simulink model "torque_est_code_source"  (R2024b)
settings: Solver=VariableStepAuto  StartTime=0.0  StopTime=20  RelTol=1e-3
model workspace (MAT data in the model file):
  Efficiency = 106.795164671
  Ktau = 0.0593933626833
  Kw = 0.000707222843993
  To = 0.029588829084
  alfa = 1.29
undefined symbols (not defined in the file or in its folder): DiscIntNeverNeededParam
settings Model: Creator=ascalzo  LastModifiedBy=upattacini
settings OptimizationCC: DefaultParameterBehavior=Inlined  UseDivisionForNetSlopeComputation=on  GainParamInheritBuiltInType=on  UseFloatMulNetSlope=on  InlineInvariantSignals=on  PassReuseOutputArgsAs=Individual arguments  ZeroExternalMemoryAtStartup=off  ZeroInternalMemoryAtStartup=off  NoFixptDivByZeroProtection=on  EfficientFloat2IntCast=on  LifeSpan=1  OptimizeBlockOrder=speed  DifferentSizesBufferReuse=on  EfficientTunableParamExpr=on
settings DebuggingCC: ParameterTunabilityLossMsg=error
settings HardwareCC: ProdBitPerPointer=32  ProdBitPerSizeT=32  ProdBitPerPtrDiffT=32  ProdLargestAtomicInteger=Long  ProdLargestAtomicFloat=Double  ProdWordSize=32  ProdLongLongMode=on  ProdHWDeviceType=ARM Compatible->ARM Cortex-M
settings SFSimCC: MATLABDynamicMemAlloc=off
settings RTWCC: Description=Embedded Coder  SystemTargetFile=ert.tlc  GenCodeOnly=on  TemplateMakefile=ert_default_tmf  TargetLang=C++  GPUComputeCapability=3.5
settings CodeAppCC: ForceParamTrailComments=on  IgnoreCustomStorageClasses=off  OperatorAnnotations=on  SimulinkDataObjDesc=on  SFDataObjDesc=on  CustomSymbolStrGlobalVar=rt$N$M  CustomSymbolStrType=$N$M  CustomSymbolStrFcn=$N$M$F  CustomSymbolStrMacro=$N$M  InsertBlockDesc=on
settings ERTTargetCC: TargetLangStandard=C++11 (ISO)  CodeReplacementLibrary=ARM Cortex-M  GenerateSampleERTMain=on  IncludeMdlTerminateFcn=off  CombineSignalStateStructs=on  CodeInterfacePackaging=C++ class  SupportComplex=off  SupportNonInlinedSFcns=on  RootIOFormat=Structure reference  ERTCustomFileTemplate=example_file_process.tlc  ERTFilePackagingFormat=CompactWithDataFile  DynamicArrayContainerType=coder::array

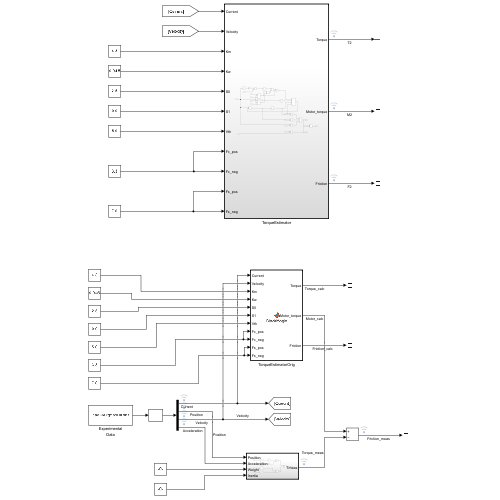
[thumbnail: Simulink's stored preview of the top-level diagram]
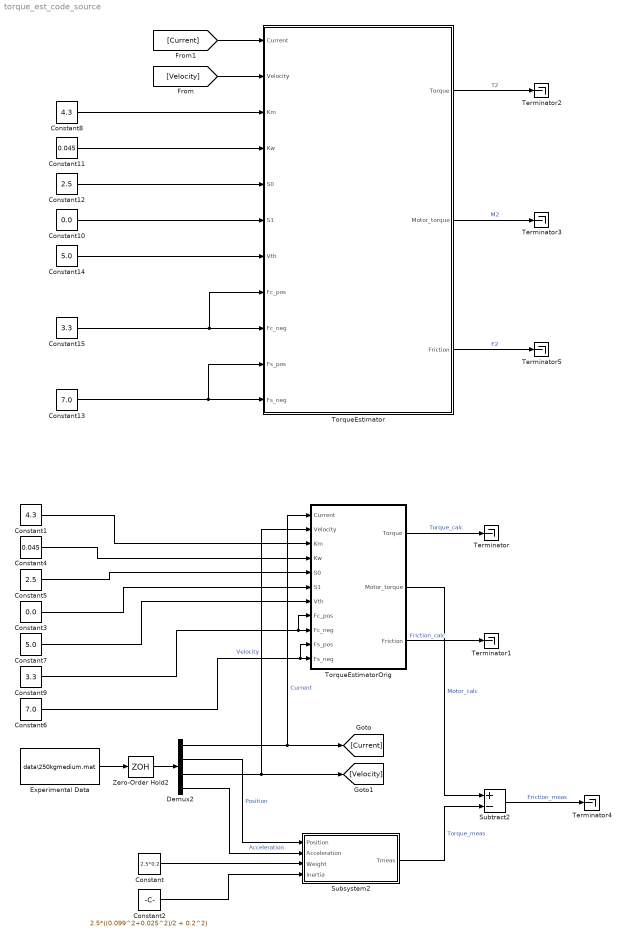
== system torque_est_code_source ==
  Constant : Constant  Value=2.5*0.2
  Constant1 : Constant  Value=4.3
  Constant10 : Constant  Value=0.0
  Constant11 : Constant  Value=0.045
  Constant12 : Constant  Value=2.5
  Constant13 : Constant  Value=7.0
  Constant14 : Constant  Value=5.0
  Constant15 : Constant  Value=3.3
  Constant2 : Constant  Value=2.5*((0.099^2+0.025^2)/2 + 0.2^2)
  Constant3 : Constant  Value=0.0
  Constant4 : Constant  Value=0.045
  Constant5 : Constant  Value=2.5
  Constant6 : Constant  Value=7.0
  Constant7 : Constant  Value=5.0
  Constant8 : Constant  Value=4.3
  Constant9 : Constant  Value=3.3
  Demux2 : Demux
  Experimental Data : FromFile  FileName=data\250kgmedium.mat  SampleTime=0.001  InterpolationWithinTimeRange=Zero order hold
  Subsystem2 : Subsystem  TreatAsAtomicUnit=on
  Subtract2 : Sum  Inputs=+-
  Terminator{,1..5} (6 alike) : Terminator
  TorqueEstimator : Subsystem  TreatAsAtomicUnit=on
  TorqueEstimatorOrig : MATLAB Function  TreatAsAtomicUnit=on
  Zero-Order Hold2 : ZeroOrderHold  SampleTime=0.001
  wires:
  Subtract2/1 -> Terminator4/1  "Friction_meas"
  Experimental Data/1 -> Zero-Order Hold2/1
  Demux2/3 -> [Velocity], TorqueEstimatorOrig/2(Velocity)  "Velocity"
  Zero-Order Hold2/1 -> Demux2/1
  Demux2/4 -> Subsystem2/2(Acceleration)  "Acceleration"
  Demux2/2 -> Subsystem2/1(Position)  "Position"
  Constant/1 -> Subsystem2/3(Weight)
  Constant2/1 -> Subsystem2/4(Inertia)
  Demux2/1 -> [Current], TorqueEstimatorOrig/1(Current)  "Current"
  Subsystem2/1(Tmeas) -> Subtract2/2  "Torque_meas"
  TorqueEstimatorOrig/2(Motor_torque) -> Subtract2/1  "Motor_calc"
  TorqueEstimatorOrig/1(Torque) -> Terminator/1  "Torque_calc"
  TorqueEstimatorOrig/3(Friction) -> Terminator1/1  "Friction_calc"
  Constant1/1 -> TorqueEstimatorOrig/3(Km)
  Constant3/1 -> TorqueEstimatorOrig/6(S1)
  Constant4/1 -> TorqueEstimatorOrig/4(Kw)
  Constant5/1 -> TorqueEstimatorOrig/5(S0)
  Constant6/1 -> TorqueEstimatorOrig/11(Fs_neg), TorqueEstimatorOrig/10(Fs_pos)
  Constant7/1 -> TorqueEstimatorOrig/7(Vth)
  Constant9/1 -> TorqueEstimatorOrig/8(Fc_pos), TorqueEstimatorOrig/9(Fc_neg)
  [Velocity] -> TorqueEstimator/2(Velocity)
  [Current] -> TorqueEstimator/1(Current)
  Constant10/1 -> TorqueEstimator/6(S1)
  Constant15/1 -> TorqueEstimator/8(Fc_pos), TorqueEstimator/9(Fc_neg)
  Constant12/1 -> TorqueEstimator/5(S0)
  Constant14/1 -> TorqueEstimator/7(Vth)
  Constant11/1 -> TorqueEstimator/4(Kw)
  Constant13/1 -> TorqueEstimator/11(Fs_neg), TorqueEstimator/10(Fs_pos)
  Constant8/1 -> TorqueEstimator/3(Km)
  TorqueEstimator/1(Torque) -> Terminator2/1  "T2"
  TorqueEstimator/2(Motor_torque) -> Terminator3/1  "M2"
  TorqueEstimator/3(Friction) -> Terminator5/1  "F2"

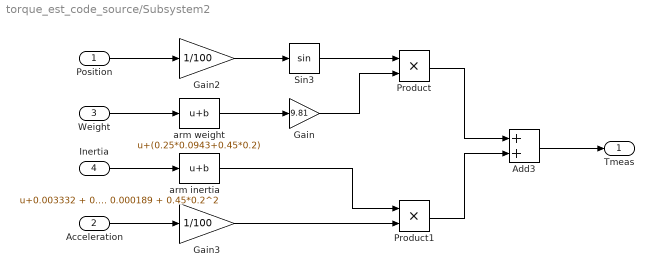
== system torque_est_code_source/Subsystem2 ==
  Position : Inport
  Acceleration : Inport  Port=2
  Weight : Inport  Port=3
  Inertia : Inport  Port=4
  Add3 : Sum
  Gain : Gain  Gain=9.81
  Gain2 : Gain  Gain=1/100
  Gain3 : Gain  Gain=1/100
  Product : Product
  Product1 : Product
  Sin3 : Trigonometry
  arm inertia : Bias  Bias=0.003332 + 0.000021 + 0.000001185 + 0.000189 + 0.45*0.2^2  SaturateOnIntegerOverflow=off
  arm weight : Bias  Bias=(0.25*0.0943+0.45*0.2)  SaturateOnIntegerOverflow=off
  Tmeas : Outport
  wires:
  Product/1 -> Add3/1
  Gain2/1 -> Sin3/1
  Sin3/1 -> Product/1
  Add3/1 -> Tmeas/1
  Gain3/1 -> Product1/2
  Acceleration/1 -> Gain3/1
  Position/1 -> Gain2/1
  Weight/1 -> arm weight/1
  Product1/1 -> Add3/2
  Inertia/1 -> arm inertia/1
  arm weight/1 -> Gain/1
  arm inertia/1 -> Product1/1
  Gain/1 -> Product/2

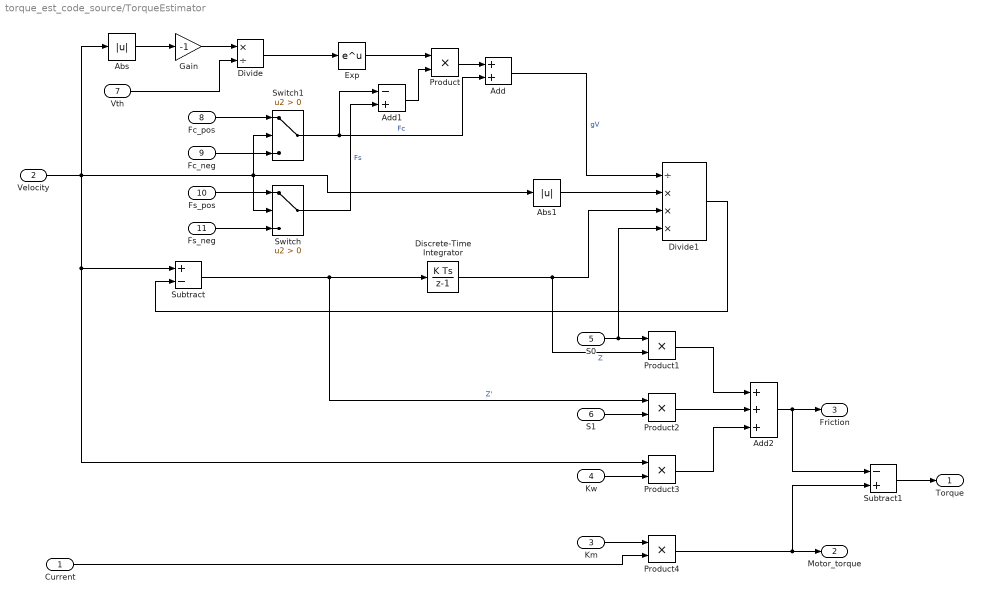
== system torque_est_code_source/TorqueEstimator ==
  Current : Inport
  Velocity : Inport  Port=2
  Km : Inport  Port=3
  Kw : Inport  Port=4
  S0 : Inport  Port=5
  S1 : Inport  Port=6
  Vth : Inport  Port=7
  Fc_pos : Inport  Port=8
  Fc_neg : Inport  Port=9
  Fs_pos : Inport  Port=10
  Fs_neg : Inport  Port=11
  Abs : Abs  SaturateOnIntegerOverflow=off
  Abs1 : Abs  SaturateOnIntegerOverflow=off
  Add : Sum
  Add1 : Sum  Inputs=-+
  Add2 : Sum  Inputs=+++
  Discrete-Time Integrator : DiscreteIntegrator  SampleTime=-1  ICPrevOutput=DiscIntNeverNeededParam  ICPrevScaledInput=DiscIntNeverNeededParam
  Divide : Product  Inputs=*/
  Divide1 : Product  Inputs=/***
  Exp : Math
  Gain : Gain  Gain=-1
  Product{,1..4} (5 alike) : Product
  Subtract : Sum  Inputs=+-
  Subtract1 : Sum  Inputs=-+
  Switch : Switch  Criteria=u2 > Threshold  SaturateOnIntegerOverflow=off  InputSameDT=off
  Switch1 : Switch  Criteria=u2 > Threshold  SaturateOnIntegerOverflow=off  InputSameDT=off
  Torque : Outport
  Motor_torque : Outport  Port=2
  Friction : Outport  Port=3
  wires:
  Fs_pos/1 -> Switch/1
  Kw/1 -> Product3/2
  Abs1/1 -> Divide1/2
  S0/1 -> Divide1/4, Product1/1
  Product2/1 -> Add2/2
  Velocity/1 -> Abs1/1, Switch/2, Switch1/2, Product3/1, Subtract/1, Abs/1
  Fs_neg/1 -> Switch/3
  Switch1/1 -> Add/2, Add1/1  "Fc"
  Subtract/1 -> Discrete-Time Integrator/1, Product2/1  "Z'"
  Exp/1 -> Product/1
  Discrete-Time Integrator/1 -> Divide1/3, Product1/2  "Z"
  Fc_neg/1 -> Switch1/3
  Fc_pos/1 -> Switch1/1
  Gain/1 -> Divide/1
  Product1/1 -> Add2/1
  Abs/1 -> Gain/1
  Product3/1 -> Add2/3
  S1/1 -> Product2/2
  Add1/1 -> Product/2
  Divide/1 -> Exp/1
  Add2/1 -> Subtract1/1, Friction/1
  Vth/1 -> Divide/2
  Product/1 -> Add/1
  Divide1/1 -> Subtract/2
  Switch/1 -> Add1/2  "Fs"
  Add/1 -> Divide1/1  "gV"
  Km/1 -> Product4/1
  Current/1 -> Product4/2
  Product4/1 -> Subtract1/2, Motor_torque/1
  Subtract1/1 -> Torque/1

== matlab function torque_est_code_source/TorqueEstimatorOrig ==
  data: Current input; Velocity input; Km input; Torque output; Motor_torque output; Friction output; Kw input; S0 input; S1 input; Vth input; Fc_pos input; Fc_neg input; Fs_pos input; Fs_neg input
function [Torque,Motor_torque,Friction] = BlackMagic(Current,Velocity,Km,Kw,S0,S1,Vth,Fc_pos,Fc_neg,Fs_pos,Fs_neg)

persistent z; % LuGre model internal state

if isempty(z)
    z = 0.0;
end

% Km = 4.3;
% Kw = 0.045;
% S0 = 2.5;
% S1 = 0.0;
% Vth = 5.0;
% Fc = 3.3;
% Fs = 7.0;

Fc = 0.0;
Fs = 0.0;

if Velocity >= 0.0
    Fc = Fc_pos;
    Fs = Fs_pos;
else
    Fc = Fc_neg;
    Fs = Fs_neg;
end

gV = Fc + (Fs-Fc)*exp(-abs(Velocity/Vth));

zdot = (Velocity - abs(Velocity)*S0*z/gV);

z = z + 0.001*zdot;

Motor_torque = Km*Current;

Friction = Kw*Velocity + S0*z + S1*zdot;

Torque = Km*Current - Kw*Velocity -S0*z - S1*zdot; %-3.3*tanh(V/10);
